simulink model "dcdc_zvs_full_bridge"  (R2026b)
settings: Solver=ode23tb  StopTime=simlength  FixedStep=tc  MaxStep=tc
values from neighbouring files (symbols this model uses):
  Idc_FS = max(Idab1_dc_nom,Idab2_dc_nom) * margin_factor    [init_model.m]
  L_core_length = 95    [magnetics_design_transformer.m]
  number_of_cells_2_sim = floor((Uout_nom-delta_load)/u_cell)    [init_model.m]    (also in run_sim_output_current_ctrl.m = floor((Uout_max-delta_load)/u_cell))
  Pnom = 175e3    (= 175000)    [init_model.m]
  tc = ts_dab/400    (= 5e-07)    [init_model.m]
  u_cell = 3.6    [init_model.m]
  Vdab2_dc_nom = ubattery2    (= 540)    [init_model.m]
  Vdc_FS = max(Vdab1_dc_nom,Vdab2_dc_nom) * margin_factor    [init_model.m]
libraries: fl_lib x32, nesl_utility x22, discrete_time_low_pass_filter x7, lithium_ion_battery x2, pi_ctrl x2, full_bridge_diode_rectifier x2, full_bridge_zvs_pwm_modulator x1, full_bridge_ideal_switch x1, full_bridge_igbt_based_with_thermal_model x1, full_bridge_mosfet_based_with_thermal_model_zvs x1, three_windings_transformer x1
(part 1 of 2)
settings Model: SimulationMode=accelerator  Creator=LTNBDA  LastModifiedBy=d.bagnara
settings SolverCC: AutoInsertRateTranBlk=on  SolverResetMethod=Robust  ZeroCrossAlgorithm=Adaptive  ZeroCrossControl=EnableAll
settings DataIOCC: DSMLogging=off  LimitDataPoints=on  MaxDataPoints=1  ReturnWorkspaceOutputs=off  SaveFormat=Array  SaveOutput=off  SaveTime=off  SignalLogging=off  SignalLoggingSaveFormat=ModelDataLogs
settings OptimizationCC: EfficientMapNaN2IntZero=off  LifeSpan=inf  MemsetInitFltsAndDblsToZero=off
settings DebuggingCC: ArithmeticOperatorsInVariantConditions=warning  FcnCallInpInsideContextMsg=warning  MergeDetectMultiDrivingBlocksExec=none  MultiTaskCondExecSysMsg=none  MultiTaskDSMMsg=warning  MultiTaskRateTransMsg=warning  SFNoUnconditionalDefaultTransitionDiag=warning  SFUnexpectedBacktrackingDiag=warning  SaveWithParameterizedLinksMsg=none  SignalResolutionControl=TryResolveAllWithWarning  SolverPrmCheckMsg=warning  StateNameClashWarn=warning  UnderspecifiedInitializationDetection=Classic
settings HardwareCC: ProdEndianess=Unspecified  ProdEqTarget=off  ProdHWDeviceType=Generic->64-bit Embedded Processor (LP64)  ProdIntDivRoundTo=Undefined  ProdLargestAtomicFloat=None  TargetEndianess=LittleEndian  TargetHWDeviceType=MATLAB Host  TargetIntDivRoundTo=Zero  TargetLongLongMode=on
settings ModelReferenceCC: PropagateSignalLabelsOutOfModel=off
settings SFSimCC: CustomCodeUndefinedFunction=UseInterfaceOnly  SimUseLocalCustomCode=off
settings RTWCC: RTWUseLocalCustomCode=off
settings CodeAppCC: StateflowObjectComments=on
settings GRTTargetCC: CombineOutputUpdateFcns=off  GRTInterface=on  TargetLangStandard=C89/C90 (ANSI)
settings ConfigComp: CovExternalEMLEnable=off  CovSaveCumulativeToWorkspaceVar=on  CovSaveSingleToWorkspaceVar=on
settings SimscapeCC: SimscapeNormalizeSystem=off  SimscapeUseEnergyAccounting=off

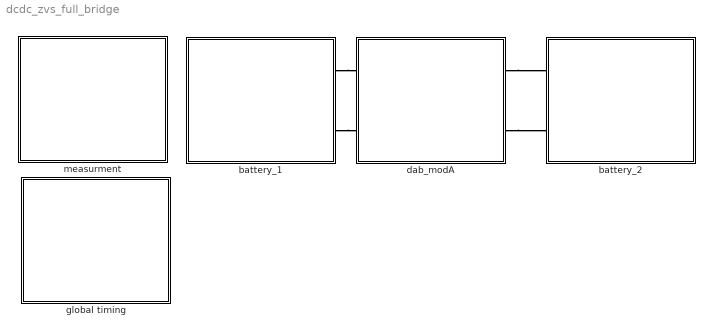
== system dcdc_zvs_full_bridge ==
  battery_1 : Subsystem
  battery_2 : Subsystem
  dab_modA : Subsystem
  global timing : Subsystem
  measurment : Subsystem
  connections:
  dab_modA/RConn2 -- battery_2/RConn2
  dab_modA/RConn1 -- battery_2/RConn1
  battery_1/RConn1 -- dab_modA/LConn1
  battery_1/RConn2 -- dab_modA/LConn2

== system dcdc_zvs_full_bridge/battery_1 ==
  Electrical Reference1 : fl_lib/Electrical/Electrical Elements/Electrical Reference
  Solver Configuration : nesl_utility/Solver Configuration  PhysicalDomain=network_engine_domain  SubClassName=solver  LeftPortType=input  RightPortType=generic  Tones=[]  Harmonics=[]  SimulateNoise=off  Profile=off  UseLocalSampling=off  EnableSwitchedLinearOptims=on  FrequencyDomain=off  UseCCode=off  RelTol=0.001  AbsTol=0.001  MinStep=1e-09  ToWorkspace=off  RevertToSquareIcSolve=off  NumHomotopyIterations=100  PhasorMode=off  PhasorModeNumHarmonics=1  ConsistencySolver=NEWTON_FTOL  CanonicalOrdering=UNORDERED  OptimizeIntermediates=UNOPTIMIZED  MulticoreSolverChoice=BACKWARD_EULER  IndexReductionMethod=DerivativeReplacement  DoDC=off  ResidualTolerance=1e-09  ConsistencyTolSource=GLOBAL  ConsistencyAbsTol=0.001  ConsistencyRelTol=0.001  ConsistencyTolFactor=0.001  UseLocalSolver=on  LocalSolverChoice=NE_BACKWARD_EULER_ADVANCER  ResolveIndetEquations=on  FunctionEvalNumThread=1  LocalSolverSampleTime=tc  DoFixedCost=on  MaxNonlinIter=5  MaxModeIter=2  ComputeImpulses=off  ImpulseIterations=2  LinearAlgebra=auto  LinearAlgebraNumThread=0  EquationFormulation=NE_TIME_EF  DelaysMemoryBudget=1024  AutomaticFiltering=on  FilteringTimeConstant=0.001  PartitionStorageMethod=AS_NEEDED  PartitionMemoryBudget=1024  PartitionMethod=BALANCED  MultibodyUseLocalSolver=off  MultibodyLocalSolverChoice=ODE1  MultibodyLocalSolverSampleTime=0.001
  litium ion battery 1 : Scope
      settings: ActiveDisplayYMinimum=741.26003825137309  ActiveDisplayYMaximum=832.30459900669575  DataLoggingVariableName=ScopeData3
  litium_ion_battery_1 : lithium_ion_battery/lithium_ion_battery  Q=Q  number_of_cells=number_of_cells_1_sim  E_1=E_1  E0=E0  E1=E1  E2=E2  E3=E3  Elog=Elog  R0=R0  R1=R1  C1=C1  M=M  alpha=alpha  soc_init=soc_init  ts_battery=ts_battery  q1Kalman=q1Kalman  q2Kalman=q2Kalman  q3Kalman=q3Kalman  rKalman=rKalman  tc=tc  enable_white_noise_m=0  battery_voltage_init_m=750
  single_phase_ui_measure : Subsystem
  dc+ : PMIOPort  Side=Right
  dc- : PMIOPort  Port=2  Side=Right
  wires:
  litium_ion_battery_1/1 -> litium ion battery 1/1
  connections:
  litium_ion_battery_1/RConn2 -- single_phase_ui_measure/LConn2 -- Electrical Reference1/LConn1 -- Solver Configuration/RConn1
  single_phase_ui_measure/RConn1 -- dc+/RConn1
  single_phase_ui_measure/LConn1 -- litium_ion_battery_1/RConn1
  dc-/RConn1 -- single_phase_ui_measure/RConn2

== system dcdc_zvs_full_bridge/battery_2 ==
  Electrical Reference1 : fl_lib/Electrical/Electrical Elements/Electrical Reference
  Resistor : fl_lib/Electrical/Electrical Elements/Resistor  Commented=on  R=(number_of_cells_2_sim*u_cell)^2/Pnom Ohm  i_specify=off  i_priority=None  i=0 A  i_nominal_specify=off  i_nominal_value=1  i_nominal_unit=A  v_specify=off  v_priority=None  v=0 V  v_nominal_specify=off  v_nominal_value=1  v_nominal_unit=V
  lithium_ion_battery_2 : lithium_ion_battery/lithium_ion_battery  Q=Q  number_of_cells=number_of_cells_2_sim  E_1=E_1  E0=E0  E1=E1  E2=E2  E3=E3  Elog=Elog  R0=R0  R1=R1  C1=C1  M=M  alpha=alpha  soc_init=soc_init  ts_battery=ts_battery  q1Kalman=q1Kalman  q2Kalman=q2Kalman  q3Kalman=q3Kalman  rKalman=rKalman  tc=tc  enable_white_noise_m=0  battery_voltage_init_m=750
  litium ion battery 2 : Scope
      settings: ActiveDisplayYMinimum=-504.55573672544915  ActiveDisplayYMaximum=-53.228038634989844  DataLoggingVariableName=ScopeData3
  single_phase_ui_measure : Subsystem
  dc+ : PMIOPort  Side=Right
  dc- : PMIOPort  Port=2  Side=Right
  wires:
  lithium_ion_battery_2/1 -> litium ion battery 2/1
  connections:
  dc-/RConn1 -- single_phase_ui_measure/RConn2
  lithium_ion_battery_2/RConn1 -- single_phase_ui_measure/LConn1 -- Resistor/LConn1
  single_phase_ui_measure/RConn1 -- dc+/RConn1
  Electrical Reference1/LConn1 -- single_phase_ui_measure/LConn2 -- Resistor/RConn1 -- lithium_ion_battery_2/RConn2

== system dcdc_zvs_full_bridge/dab_modA ==
  dab_ctrl : Subsystem
  dcdc_with_galvanic_isolation : Subsystem
  udc(+) : PMIOPort  Side=Right
  udc(-) : PMIOPort  Port=2  Side=Right
  dc+ : PMIOPort  Port=3  Side=Left
  dc- : PMIOPort  Port=4  Side=Left
  wires:
  dab_ctrl/1(gate_commands) -> dcdc_with_galvanic_isolation/1(gate_commands)
  connections:
  udc(+)/RConn1 -- dcdc_with_galvanic_isolation/RConn1
  udc(-)/RConn1 -- dcdc_with_galvanic_isolation/RConn2
  dc-/RConn1 -- dcdc_with_galvanic_isolation/LConn2
  dc+/RConn1 -- dcdc_with_galvanic_isolation/LConn1

== system dcdc_zvs_full_bridge/global timing ==
  Unit Delay : UnitDelay  SampleTime=tc
  time_afe1 : Subsystem  mask{k=1}
      mask prompts: k "Time Gain"
      mask Display:
      | disp('time-gen');
      | port_label('input', 1, 'crt');
      | port_label('output', 1, 'tout');
  time_afe3 : Subsystem  mask{k=1}
      mask prompts: k "Time Gain"
      mask Display:
      | disp('time-gen');
      | port_label('output', 1, 'tout');
  tag scope: time_dab_module_1=global, time_master=global
  wires:
  time_afe1/1(Out1) -> [time_dab_module_1]
  time_afe3/1(Out1) -> [time_master]
  [local_time_corr_dcdc1] -> Unit Delay/1
  Unit Delay/1 -> time_afe1/1(correction_time)

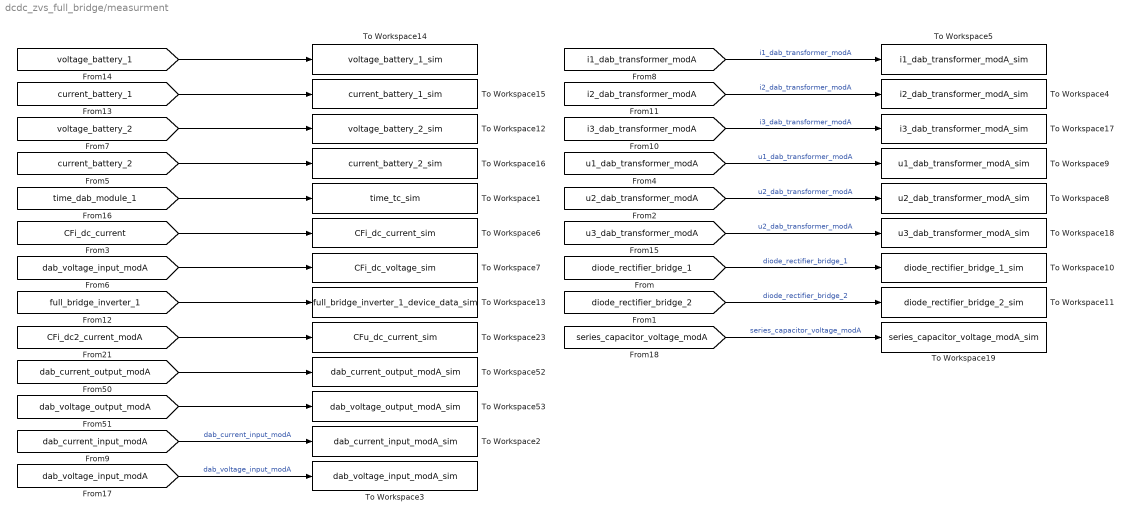
== system dcdc_zvs_full_bridge/measurment ==
  To Workspace1 : ToWorkspace  VariableName=time_tc_sim  SampleTime=tc
      settings: MaxDataPoints=Nc
  To Workspace10 : ToWorkspace  VariableName=diode_rectifier_bridge_1_sim  SampleTime=tc
      settings: MaxDataPoints=Nc
  To Workspace11 : ToWorkspace  VariableName=diode_rectifier_bridge_2_sim  SampleTime=tc
      settings: MaxDataPoints=Nc
  To Workspace12 : ToWorkspace  VariableName=voltage_battery_2_sim  SampleTime=tc
      settings: MaxDataPoints=Nc
  To Workspace13 : ToWorkspace  VariableName=full_bridge_inverter_1_device_data_sim  SampleTime=tc
      settings: MaxDataPoints=Nc
  To Workspace14 : ToWorkspace  VariableName=voltage_battery_1_sim  SampleTime=tc
      settings: MaxDataPoints=Nc
  To Workspace15 : ToWorkspace  VariableName=current_battery_1_sim  SampleTime=tc
      settings: MaxDataPoints=Nc
  To Workspace16 : ToWorkspace  VariableName=current_battery_2_sim  SampleTime=tc
      settings: MaxDataPoints=Nc
  To Workspace17 : ToWorkspace  VariableName=i3_dab_transformer_modA_sim  SampleTime=tc
      settings: MaxDataPoints=Nc
  To Workspace18 : ToWorkspace  VariableName=u3_dab_transformer_modA_sim  SampleTime=tc
      settings: MaxDataPoints=Nc
  To Workspace19 : ToWorkspace  VariableName=series_capacitor_voltage_modA_sim  SampleTime=tc
      settings: MaxDataPoints=Nc
  To Workspace2 : ToWorkspace  VariableName=dab_current_input_modA_sim  SampleTime=tc
      settings: MaxDataPoints=Nc
  To Workspace23 : ToWorkspace  VariableName=CFu_dc_current_sim  SampleTime=tc
      settings: MaxDataPoints=Nc
  To Workspace3 : ToWorkspace  VariableName=dab_voltage_input_modA_sim  SampleTime=tc
      settings: MaxDataPoints=Nc
  To Workspace4 : ToWorkspace  VariableName=i2_dab_transformer_modA_sim  SampleTime=tc
      settings: MaxDataPoints=Nc
  To Workspace5 : ToWorkspace  VariableName=i1_dab_transformer_modA_sim  SampleTime=tc
      settings: MaxDataPoints=Nc
  To Workspace52 : ToWorkspace  VariableName=dab_current_output_modA_sim  SampleTime=tc
      settings: MaxDataPoints=Nc
  To Workspace53 : ToWorkspace  VariableName=dab_voltage_output_modA_sim  SampleTime=tc
      settings: MaxDataPoints=Nc
  To Workspace6 : ToWorkspace  VariableName=CFi_dc_current_sim  SampleTime=tc
      settings: MaxDataPoints=Nc
  To Workspace7 : ToWorkspace  VariableName=CFi_dc_voltage_sim  SampleTime=tc
      settings: MaxDataPoints=Nc
  To Workspace8 : ToWorkspace  VariableName=u2_dab_transformer_modA_sim  SampleTime=tc
      settings: MaxDataPoints=Nc
  To Workspace9 : ToWorkspace  VariableName=u1_dab_transformer_modA_sim  SampleTime=tc
      settings: MaxDataPoints=Nc
  wires:
  [time_dab_module_1] -> To Workspace1/1
  [CFi_dc_current] -> To Workspace6/1
  [dab_voltage_input_modA] -> To Workspace7/1
  [voltage_battery_1] -> To Workspace14/1
  [current_battery_1] -> To Workspace15/1
  [CFi_dc2_current_modA] -> To Workspace23/1
  [dab_voltage_output_modA] -> To Workspace53/1
  [dab_current_output_modA] -> To Workspace52/1
  [full_bridge_inverter_1] -> To Workspace13/1
  [dab_current_input_modA] -> To Workspace2/1  "dab_current_input_modA"
  [dab_voltage_input_modA] -> To Workspace3/1  "dab_voltage_input_modA"
  [i2_dab_transformer_modA] -> To Workspace4/1  "i2_dab_transformer_modA"
  [i1_dab_transformer_modA] -> To Workspace5/1  "i1_dab_transformer_modA"
  [u2_dab_transformer_modA] -> To Workspace8/1  "u2_dab_transformer_modA"
  [u1_dab_transformer_modA] -> To Workspace9/1  "u1_dab_transformer_modA"
  [voltage_battery_2] -> To Workspace12/1
  [current_battery_2] -> To Workspace16/1
  [diode_rectifier_bridge_1] -> To Workspace10/1  "diode_rectifier_bridge_1"
  [diode_rectifier_bridge_2] -> To Workspace11/1  "diode_rectifier_bridge_2"
  [i3_dab_transformer_modA] -> To Workspace17/1  "i3_dab_transformer_modA"
  [u3_dab_transformer_modA] -> To Workspace18/1  "u2_dab_transformer_modA"
  [series_capacitor_voltage_modA] -> To Workspace19/1  "series_capacitor_voltage_modA"

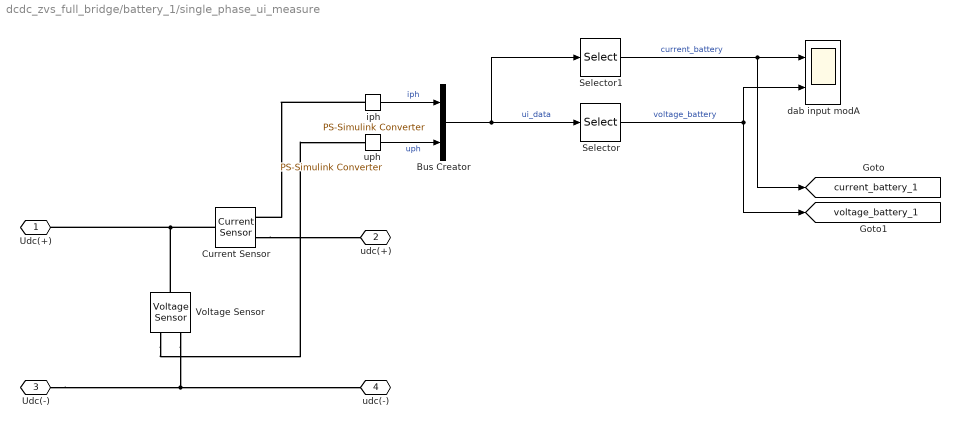
== system dcdc_zvs_full_bridge/battery_1/single_phase_ui_measure ==
  Bus Creator : BusCreator  Inputs=2
  Current Sensor : fl_lib/Electrical/Electrical Sensors/Current Sensor
  Selector : Selector  InputPortWidth=2  IndexOptions=Index vector (dialog)  Indices=2  OutputSizes=1  RuntimeRangeChecks=off
  Selector1 : Selector  InputPortWidth=2  IndexOptions=Index vector (dialog)  Indices=1  OutputSizes=1  RuntimeRangeChecks=off
  Voltage Sensor : fl_lib/Electrical/Electrical Sensors/Voltage Sensor
  dab input modA : Scope  NumInputPorts=2
      settings: SampleTime=tc  ActiveDisplayYMinimum=-4428.9106738971032  ActiveDisplayYMaximum=4853.7975894934307  DataLoggingVariableName=ScopeData2
  iph : nesl_utility/PS-Simulink Converter  PhysicalDomain=network_engine_domain  SubClassName=ps_output  LeftPortType=input  RightPortType=output  PseudoPeriodic=off  Frequencies=[]  VectorFormat=1-D array  Unit=A  AffineConversion=off
  uph : nesl_utility/PS-Simulink Converter  PhysicalDomain=network_engine_domain  SubClassName=ps_output  LeftPortType=input  RightPortType=output  PseudoPeriodic=off  Frequencies=[]  VectorFormat=1-D array  Unit=V  AffineConversion=off
  Udc(+) : PMIOPort  Side=Left
  udc(+) : PMIOPort  Port=2  Side=Right
  Udc(-) : PMIOPort  Port=3  Side=Left
  udc(-) : PMIOPort  Port=4  Side=Right
  tag scope: current_battery_1=global, voltage_battery_1=global
  wires:
  Bus Creator/1 -> Selector/1, Selector1/1  "ui_data"
  iph/1 -> Bus Creator/1  "iph"
  uph/1 -> Bus Creator/2  "uph"
  Selector1/1 -> [current_battery_1], dab input modA/1  "current_battery"
  Selector/1 -> dab input modA/2, [voltage_battery_1]  "voltage_battery"
  connections:
  iph/LConn1 -- Current Sensor/RConn1
  Voltage Sensor/LConn1 -- Current Sensor/LConn1 -- Udc(+)/RConn1
  Current Sensor/RConn2 -- udc(+)/RConn1
  Voltage Sensor/RConn1 -- uph/LConn1
  Voltage Sensor/RConn2 -- Udc(-)/RConn1 -- udc(-)/RConn1

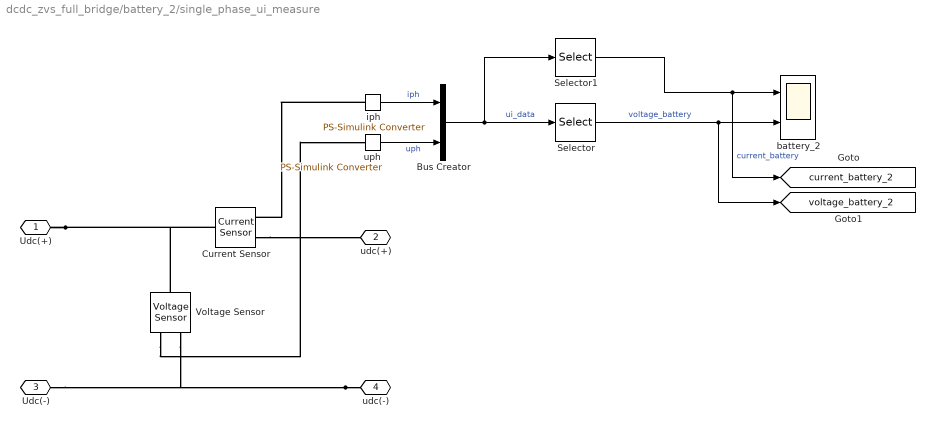
== system dcdc_zvs_full_bridge/battery_2/single_phase_ui_measure ==
  Bus Creator : BusCreator  Inputs=2
  Current Sensor : fl_lib/Electrical/Electrical Sensors/Current Sensor
  Selector : Selector  InputPortWidth=2  IndexOptions=Index vector (dialog)  Indices=2  OutputSizes=1  RuntimeRangeChecks=off
  Selector1 : Selector  InputPortWidth=2  IndexOptions=Index vector (dialog)  Indices=1  OutputSizes=1  RuntimeRangeChecks=off
  Voltage Sensor : fl_lib/Electrical/Electrical Sensors/Voltage Sensor
  battery_2 : Scope  NumInputPorts=2
      settings: SampleTime=tc  ActiveDisplayYMinimum=-384.09444656466405  ActiveDisplayYMaximum=-245.67258584008431  DataLoggingVariableName=ScopeData2
  iph : nesl_utility/PS-Simulink Converter  PhysicalDomain=network_engine_domain  SubClassName=ps_output  LeftPortType=input  RightPortType=output  PseudoPeriodic=off  Frequencies=[]  VectorFormat=1-D array  Unit=A  AffineConversion=off
  uph : nesl_utility/PS-Simulink Converter  PhysicalDomain=network_engine_domain  SubClassName=ps_output  LeftPortType=input  RightPortType=output  PseudoPeriodic=off  Frequencies=[]  VectorFormat=1-D array  Unit=V  AffineConversion=off
  Udc(+) : PMIOPort  Side=Left
  udc(+) : PMIOPort  Port=2  Side=Right
  Udc(-) : PMIOPort  Port=3  Side=Left
  udc(-) : PMIOPort  Port=4  Side=Right
  tag scope: current_battery_2=global, voltage_battery_2=global
  wires:
  Selector/1 -> [voltage_battery_2], battery_2/2  "voltage_battery"
  Selector1/1 -> battery_2/1, [current_battery_2]  "current_battery"
  uph/1 -> Bus Creator/2  "uph"
  iph/1 -> Bus Creator/1  "iph"
  Bus Creator/1 -> Selector1/1, Selector/1  "ui_data"
  connections:
  udc(-)/RConn1 -- Udc(-)/RConn1 -- Voltage Sensor/RConn2
  Voltage Sensor/RConn1 -- uph/LConn1
  Current Sensor/RConn2 -- udc(+)/RConn1
  Udc(+)/RConn1 -- Current Sensor/LConn1 -- Voltage Sensor/LConn1
  iph/LConn1 -- Current Sensor/RConn1

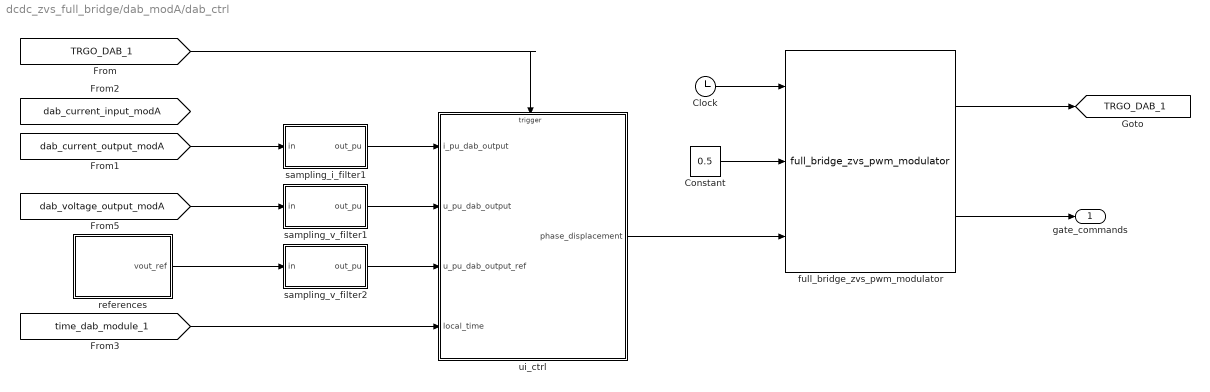
== system dcdc_zvs_full_bridge/dab_modA/dab_ctrl ==
  Clock : Clock
  Constant : Constant  Value=0.5
  full_bridge_zvs_pwm_modulator : full_bridge_zvs_pwm_modulator/full_bridge_zvs_pwm_modulator  fPWM_m=fPWM_DAB  m_up_m=1  m_low_m=0  dead_time_DAB_m=dead_time_DAB  pos_cmd_gate_m=15  neg_cmd_gate_m=-10  polarity_m=1  tc_m=tc  max_phase_displacement_m=pi  trgo_double_update_m=TRGO_double_update
  references : Subsystem
  sampling_i_filter1 : Subsystem
  sampling_v_filter1 : Subsystem
  sampling_v_filter2 : Subsystem
  ui_ctrl : Subsystem
  gate_commands : Outport
  tag scope: TRGO_DAB_1=global
  wires:
  [dab_voltage_output_modA] -> sampling_v_filter1/1(in)
  sampling_i_filter1/1(out_pu) -> ui_ctrl/1(i_pu_dab_output)
  sampling_v_filter1/1(out_pu) -> ui_ctrl/2(u_pu_dab_output)
  sampling_v_filter2/1(out_pu) -> ui_ctrl/3(u_pu_dab_output_ref)
  references/1(vout_ref) -> sampling_v_filter2/1(in)
  full_bridge_zvs_pwm_modulator/2 -> gate_commands/1
  Clock/1 -> full_bridge_zvs_pwm_modulator/1
  full_bridge_zvs_pwm_modulator/1 -> [TRGO_DAB_1]
  [TRGO_DAB_1] -> ui_ctrl/Trigger
  Constant/1 -> full_bridge_zvs_pwm_modulator/2
  ui_ctrl/1(phase_displacement) -> full_bridge_zvs_pwm_modulator/3
  [dab_current_output_modA] -> sampling_i_filter1/1(in)
  [time_dab_module_1] -> ui_ctrl/4(local_time)

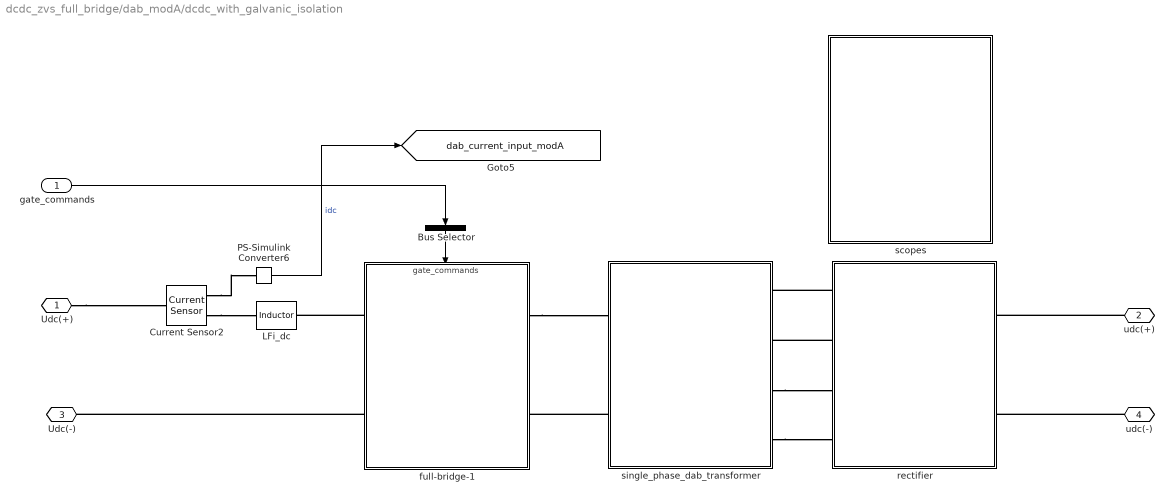
== system dcdc_zvs_full_bridge/dab_modA/dcdc_with_galvanic_isolation ==
  gate_commands : Inport
  Bus Selector : BusSelector  OutputSignals=gate_cmd_Q1,gate_cmd_Q2,gate_cmd_Q3,gate_cmd_Q4  OutputAsBus=on
  Current Sensor2 : fl_lib/Electrical/Electrical Sensors/Current Sensor
  LFi_dc : fl_lib/Electrical/Electrical Elements/Inductor  l=LFi_dc H  r=RLFi_dc Ohm  g=1e-9 1/Ohm  i_specify=off  i_priority=None  i=0 A  i_nominal_specify=off  i_nominal_value=1  i_nominal_unit=A  v_specify=off  v_priority=None  v=0 V  v_nominal_specify=off  v_nominal_value=1  v_nominal_unit=V  i_L_specify=off  i_L_priority=High  i_L=0 A  i_L_nominal_specify=off  i_L_nominal_value=1  i_L_nominal_unit=A
  PS-Simulink Converter6 : nesl_utility/PS-Simulink Converter  PhysicalDomain=network_engine_domain  SubClassName=ps_output  LeftPortType=input  RightPortType=output  PseudoPeriodic=off  Frequencies=[]  VectorFormat=1-D array  Unit=A  AffineConversion=on
  full-bridge-1 : Subsystem
      settings: PortSchema="{\"entries\":[{\"content\":{\"sides\":[{\"content\":{\"connectorIds\":[\"LConn1\",\"LConn2\"]},\"type\":\"ConnectorPlacement.EquallySpacedRectSide\",\"uuid\":\"c872503a-61af-4937-bdf2-4de4f8645573\"},{\"content\":{\"connectorIds\":[\"RConn1\",\"RConn2\"],\"side\":\"RIGHT\"},\"type\":\"ConnectorPlacement.EquallySpacedRectSide\",\"uuid\":\"3b83f060-86a2-4569-84b5-d9f7c0485347\"},{\"content\":{\"connectorIds\":[\"In1\"],\"side\":\"TOP\"},\"type\":\"ConnectorPlacement.EquallySpacedRectSide\",\"uuid\":\"bf191d46-ce71-4d15-9dd0-24cc57253577\"}]},\"type\":\"ConnectorPlacement.EquallySpacedConnector\",\"uuid\":\"1b28ceee-25d0-45ae-a3c4-c2563f0d63ba\"}],\"packageUris\":[\"http://schema.mathworks.com/mf0/Connector/R2020b\"],\"version\":\"1.0\"}"
  rectifier : Subsystem
  scopes : Subsystem
  single_phase_dab_transformer : Subsystem
  Udc(+) : PMIOPort  Side=Left
  udc(+) : PMIOPort  Port=2  Side=Right
  Udc(-) : PMIOPort  Port=3  Side=Left
  udc(-) : PMIOPort  Port=4  Side=Right
  tag scope: dab_current_input_modA=global
  wires:
  gate_commands/1 -> Bus Selector/1
  PS-Simulink Converter6/1 -> [dab_current_input_modA]  "idc"
  Bus Selector/1 -> full-bridge-1/1(gate_commands)
  connections:
  single_phase_dab_transformer/LConn2 -- full-bridge-1/LConn2
  full-bridge-1/RConn1 -- LFi_dc/RConn1
  full-bridge-1/RConn2 -- Udc(-)/RConn1
  full-bridge-1/LConn1 -- single_phase_dab_transformer/LConn1
  udc(-)/RConn1 -- rectifier/RConn2
  Current Sensor2/RConn2 -- LFi_dc/LConn1
  Udc(+)/RConn1 -- Current Sensor2/LConn1
  Current Sensor2/RConn1 -- PS-Simulink Converter6/LConn1
  rectifier/LConn1 -- single_phase_dab_transformer/RConn1
  rectifier/LConn2 -- single_phase_dab_transformer/RConn2
  udc(+)/RConn1 -- rectifier/RConn1
  single_phase_dab_transformer/RConn3 -- rectifier/LConn3
  single_phase_dab_transformer/RConn4 -- rectifier/LConn4

== system dcdc_zvs_full_bridge/global timing/time_afe1 ==
  correction_time : Inport
  Constant : Constant
  Gain : Gain  Gain=k
  Product : Product
  Sum : Sum  Inputs=|++
  time_1 : Clock
  Out1 : Outport
  wires:
  time_1/1 -> Gain/1
  Gain/1 -> Product/1
  Product/1 -> Out1/1
  correction_time/1 -> Sum/1
  Sum/1 -> Product/2
  Constant/1 -> Sum/2

== system dcdc_zvs_full_bridge/global timing/time_afe3 ==
  Gain : Gain  Gain=k
  time_1 : Clock
  Out1 : Outport
  wires:
  Gain/1 -> Out1/1
  time_1/1 -> Gain/1

== system dcdc_zvs_full_bridge/dab_modA/dab_ctrl/references ==
  Rate Limiter : RateLimiter  RisingSlewLimit=Vdab2_dc_nom*10  FallingSlewLimit=-Vdab2_dc_nom*10  SampleTimeMode=inherited
  Vout_dc_nom : Step  Time=1e-3  FinalValue=Vdab2_dc_nom  SampleTime=0
  vout_ref : Outport
  wires:
  Rate Limiter/1 -> vout_ref/1
  Vout_dc_nom/1 -> Rate Limiter/1

== system dcdc_zvs_full_bridge/dab_modA/dab_ctrl/sampling_i_filter1 ==
  in : Inport
  1/Ti3 : Gain  Gain=1/Idc_FS  OutDataTypeStr=double  SaturateOnIntegerOverflow=on  ParamDataTypeStr=Inherit: Same as input
  out_pu : Outport
  wires:
  in/1 -> 1/Ti3/1
  1/Ti3/1 -> out_pu/1

== system dcdc_zvs_full_bridge/dab_modA/dab_ctrl/sampling_v_filter1 ==
  in : Inport
  1/Ti3 : Gain  Gain=1/Vdc_FS  OutDataTypeStr=double  SaturateOnIntegerOverflow=on  ParamDataTypeStr=Inherit: Same as input
  out_pu : Outport
  wires:
  in/1 -> 1/Ti3/1
  1/Ti3/1 -> out_pu/1

== system dcdc_zvs_full_bridge/dab_modA/dab_ctrl/sampling_v_filter2 ==
  in : Inport
  1/Ti3 : Gain  Gain=1/Vdc_FS  OutDataTypeStr=double  SaturateOnIntegerOverflow=on  ParamDataTypeStr=Inherit: Same as input
  Saturation : Saturate  UpperLimit=1  LowerLimit=0  OutDataTypeStr=double
  out_pu : Outport
  wires:
  in/1 -> 1/Ti3/1
  1/Ti3/1 -> Saturation/1
  Saturation/1 -> out_pu/1

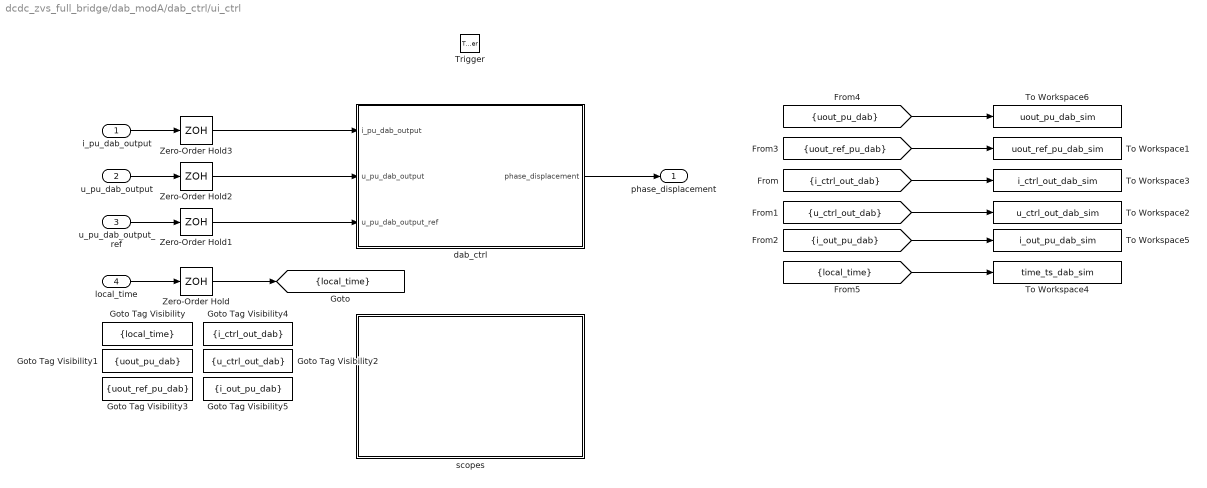
== system dcdc_zvs_full_bridge/dab_modA/dab_ctrl/ui_ctrl ==
  i_pu_dab_output : Inport
  u_pu_dab_output : Inport  Port=2
  u_pu_dab_output_ref : Inport  Port=3
  local_time : Inport  Port=4
  Trigger : TriggerPort  VariantControl=(inherit)  PortDimensions=1
  Goto Tag Visibility : GotoTagVisibility  GotoTag=local_time
  Goto Tag Visibility1 : GotoTagVisibility  GotoTag=uout_pu_dab
  Goto Tag Visibility2 : GotoTagVisibility  GotoTag=u_ctrl_out_dab
  Goto Tag Visibility3 : GotoTagVisibility  GotoTag=uout_ref_pu_dab
  Goto Tag Visibility4 : GotoTagVisibility  GotoTag=i_ctrl_out_dab
  Goto Tag Visibility5 : GotoTagVisibility  GotoTag=i_out_pu_dab
  To Workspace1 : ToWorkspace  VariableName=uout_ref_pu_dab_sim  SampleTime=-1
      settings: MaxDataPoints=Ns_dab
  To Workspace2 : ToWorkspace  VariableName=u_ctrl_out_dab_sim  SampleTime=-1
      settings: MaxDataPoints=Ns_dab
  To Workspace3 : ToWorkspace  VariableName=i_ctrl_out_dab_sim  SampleTime=-1
      settings: MaxDataPoints=Ns_dab
  To Workspace4 : ToWorkspace  VariableName=time_ts_dab_sim  SampleTime=-1
      settings: MaxDataPoints=Ns_dab
  To Workspace5 : ToWorkspace  VariableName=i_out_pu_dab_sim  SampleTime=-1
      settings: MaxDataPoints=Ns_dab
  To Workspace6 : ToWorkspace  VariableName=uout_pu_dab_sim  SampleTime=-1
      settings: MaxDataPoints=Ns_dab
  Zero-Order Hold{,1..3} (4 alike) : ZeroOrderHold  SampleTime=-1
  dab_ctrl : Subsystem
  scopes : Subsystem
  phase_displacement : Outport
  tag scope: local_time=scoped
  wires:
  i_pu_dab_output/1 -> Zero-Order Hold3/1
  u_pu_dab_output/1 -> Zero-Order Hold2/1
  u_pu_dab_output_ref/1 -> Zero-Order Hold1/1
  dab_ctrl/1(phase_displacement) -> phase_displacement/1
  local_time/1 -> Zero-Order Hold/1
  Zero-Order Hold1/1 -> dab_ctrl/3(u_pu_dab_output_ref)
  Zero-Order Hold2/1 -> dab_ctrl/2(u_pu_dab_output)
  Zero-Order Hold3/1 -> dab_ctrl/1(i_pu_dab_output)
  Zero-Order Hold/1 -> [local_time]
  [uout_ref_pu_dab] -> To Workspace1/1
  [uout_pu_dab] -> To Workspace6/1
  [u_ctrl_out_dab] -> To Workspace2/1
  [i_ctrl_out_dab] -> To Workspace3/1
  [local_time] -> To Workspace4/1
  [i_out_pu_dab] -> To Workspace5/1

== system dcdc_zvs_full_bridge/dab_modA/dcdc_with_galvanic_isolation/full-bridge-1 ==
  gate_commands : Inport
  dclink : Subsystem
  full-bridge ideal switch based : full_bridge_ideal_switch/full-bridge ideal switch based  Commented=on  Rds_on=Rds_on  Vdon_diode=Vdon_diode  Rdon_diode=Rdon_diode  Csnubber=Csnubber  Rsnubber=Rsnubber  Vth=Vth
  full-bridge-igbt-based-with-thermal-model : full_bridge_igbt_based_with_thermal_model/full-bridge-igbt-based-with-thermal-model  mass_heatsink_m=heatsink.no_weight  specific_heat_m=heatsink.cp  rth_mosfet_HA_m=heatsink.Rth_switch_HA  rth_mosfet_JH_m=dab.igbt.Rth_switch_JH  Rce_on_m=dab.igbt.Rce_on  Vce_sat_m=dab.igbt.Vce_sat  Vth_m=dab.igbt.Vth  Eon_m=dab.igbt.Eon  Eoff_m=dab.igbt.Eoff  Erec_m=dab.igbt.Erec  Voff_sw_loss_m=dab.igbt.Voff_sw_losses  Ion_sw_loss_m=dab.igbt.Ion_sw_losses  Vdon_diode_m=dab.igbt.Vdon_diode  Rdon_diode_m=dab.igbt.Rdon_diode  Csnubber_m=dab.igbt.Csnubber  Rsnubber_m=dab.igbt.Rsnubber  JunctionTermalMass_m=dab.igbt.JunctionTermalMass  Tambient_m=Tambient  DThs_init_m=DThs_init  filter_time_constant_m=dab.igbt.filter_time_constant  tc_m=tc
  full-bridge_mosfet_based_ with_thermal_model_zvs : full_bridge_mosfet_based_with_thermal_model_zvs/full-bridge_mosfet_based_ with_thermal_model_zvs  Commented=on  mass_heatsink_m=weigth  specific_heat_m=cp_al  rth_mosfet_HA_m=Rth_mosfet_HA  rth_mosfet_JH_m=dab_mosfet.Rth_mosfet_JH  Rds_on_m=dab_mosfet.Rds_on  Vth_m=dab_mosfet.Vth  Eon_m=dab_mosfet.Eon  Eoff_m=dab_mosfet.Eoff  Voff_sw_loss_m=dab_mosfet.Voff_sw_losses  Ion_sw_loss_m=dab_mosfet.Ion_sw_losses  Vdon_diode_m=dab_mosfet.Vdon_diode  Rdon_diode_m=dab_mosfet.Rdon_diode  JunctionTermalMass_m=dab_mosfet.JunctionTermalMass  Tambient_m=Tambient  DThs_init_m=DThs_init  Csnubber_m=dab_mosfet.Csnubber_zvs  Rsnubber_m=dab_mosfet.Rsnubber_zvs
  uac_1(+) : PMIOPort  Side=Left
  uac_1(-) : PMIOPort  Port=2  Side=Left
  Udc(+) : PMIOPort  Port=3  Side=Right
  Udc(-) : PMIOPort  Port=4  Side=Right
  tag scope: full_bridge_inverter_1=global
  wires:
  gate_commands/1 -> full-bridge ideal switch based/1, full-bridge-igbt-based-with-thermal-model/1, full-bridge_mosfet_based_ with_thermal_model_zvs/1
  full-bridge-igbt-based-with-thermal-model/1 -> [full_bridge_inverter_1]
  connections:
  uac_1(+)/RConn1 -- full-bridge_mosfet_based_ with_thermal_model_zvs/RConn1 -- full-bridge-igbt-based-with-thermal-model/RConn1 -- full-bridge ideal switch based/RConn1
  uac_1(-)/RConn1 -- full-bridge_mosfet_based_ with_thermal_model_zvs/RConn2 -- full-bridge-igbt-based-with-thermal-model/RConn2 -- full-bridge ideal switch based/RConn2
  dclink/LConn1 -- Udc(+)/RConn1
  dclink/RConn2 -- full-bridge ideal switch based/LConn2 -- full-bridge_mosfet_based_ with_thermal_model_zvs/LConn2 -- full-bridge-igbt-based-with-thermal-model/LConn2
  dclink/RConn1 -- full-bridge_mosfet_based_ with_thermal_model_zvs/LConn1 -- full-bridge-igbt-based-with-thermal-model/LConn1 -- full-bridge ideal switch based/LConn1
  dclink/LConn2 -- Udc(-)/RConn1

== system dcdc_zvs_full_bridge/dab_modA/dcdc_with_galvanic_isolation/rectifier ==
  dclink : Subsystem
  rectifier_1 : Subsystem
  rectifier_2 : Subsystem
  uac_2(+) : PMIOPort  Side=Left
  uac_2(-) : PMIOPort  Port=2  Side=Left
  udc(+) : PMIOPort  Port=3  Side=Right
  udc(-) : PMIOPort  Port=4  Side=Right
  uac_3(+) : PMIOPort  Port=5  Side=Left
  uac_3(-) : PMIOPort  Port=6  Side=Left
  connections:
  udc(+)/RConn1 -- dclink/RConn1
  udc(-)/RConn1 -- dclink/RConn2
  uac_2(+)/RConn1 -- rectifier_1/LConn1
  dclink/LConn1 -- rectifier_1/RConn1
  uac_2(-)/RConn1 -- rectifier_1/LConn2
  rectifier_2/LConn2 -- uac_3(-)/RConn1
  rectifier_2/LConn1 -- uac_3(+)/RConn1
  rectifier_1/RConn2 -- rectifier_2/RConn1
  rectifier_2/RConn2 -- dclink/LConn2

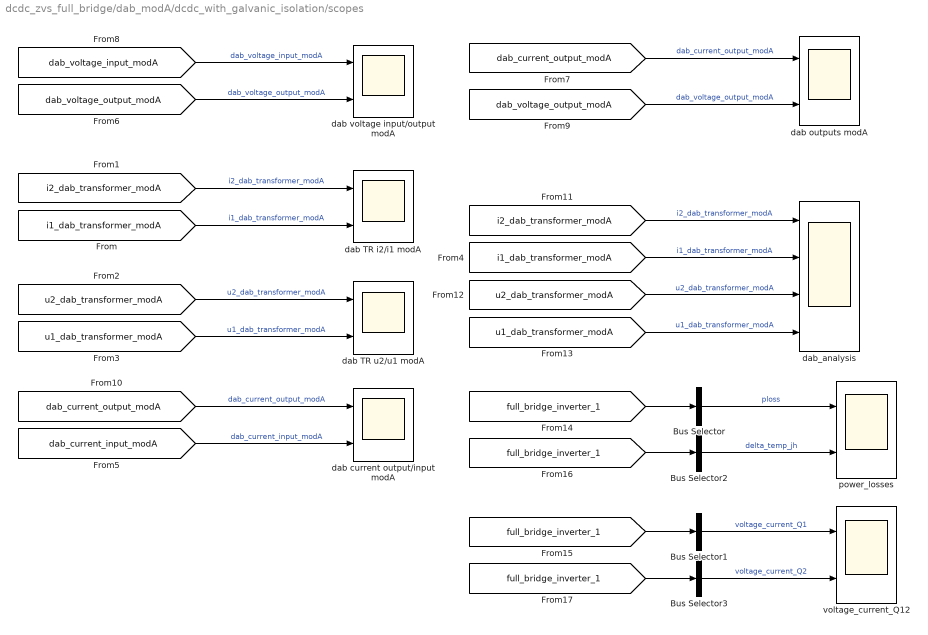
== system dcdc_zvs_full_bridge/dab_modA/dcdc_with_galvanic_isolation/scopes ==
  Bus Selector : BusSelector  OutputSignals=igbt_ploss_Q1,igbt_ploss_Q2,igbt_ploss_Q3,igbt_ploss_Q4  OutputAsBus=on
  Bus Selector1 : BusSelector  OutputSignals=igbt_voltage_Q1,igbt_current_Q1  OutputAsBus=on
  Bus Selector2 : BusSelector  OutputSignals=igbt_JH_temp_Q1,igbt_JH_temp_Q4,igbt_JH_temp_Q3,igbt_JH_temp_Q2  OutputAsBus=on
  Bus Selector3 : BusSelector  OutputSignals=igbt_voltage_Q2,igbt_current_Q2  OutputAsBus=on
  dab TR i2/i1 modA : Scope  NumInputPorts=2
      settings: SampleTime=tc  ActiveDisplayYMinimum=-1133.8385972087863  ActiveDisplayYMaximum=1130.02633442417  DataLoggingVariableName=ScopeData13
  dab TR u2/u1 modA : Scope  NumInputPorts=2
      settings: SampleTime=tc  ActiveDisplayYMinimum=-1550.0820677220172  ActiveDisplayYMaximum=1550.0802549877285  DataLoggingVariableName=ScopeData4
  dab current output/input modA : Scope  NumInputPorts=2
      settings: SampleTime=tc  ActiveDisplayYMinimum=-135.33312051034864  ActiveDisplayYMaximum=747.30464050791215  DataLoggingVariableName=ScopeData8
  dab outputs modA : Scope  NumInputPorts=2
      settings: SampleTime=tc  ActiveDisplayYMinimum=-176.23009288903958  ActiveDisplayYMaximum=438.21126312258008  DataLoggingVariableName=ScopeData6
  dab voltage input/output modA : Scope  NumInputPorts=2
      settings: SampleTime=tc  ActiveDisplayYMinimum=-220.62176138017153  ActiveDisplayYMaximum=1985.59585243125  DataLoggingVariableName=ScopeData10
  dab_analysis : Scope  NumInputPorts=4
      settings: SampleTime=tc  ActiveDisplayYMinimum=-3557.7801563621397  ActiveDisplayYMaximum=1974.1341111521624  DataLoggingVariableName=ScopeData5
  power_losses : Scope  NumInputPorts=2
      settings: SampleTime=tc  ActiveDisplayYMinimum=-425.00761228440524  ActiveDisplayYMaximum=-42.577893314830831
  voltage_current_Q12 : Scope  NumInputPorts=2
      settings: SampleTime=tc  ActiveDisplayYMinimum=251.19059945367908  ActiveDisplayYMaximum=349.10358624180844  DataLoggingVariableName=ScopeData14
  wires:
  [dab_voltage_input_modA] -> dab voltage input/output modA/1  "dab_voltage_input_modA"
  [dab_current_output_modA] -> dab current output/input modA/1  "dab_current_output_modA"
  [dab_voltage_output_modA] -> dab voltage input/output modA/2  "dab_voltage_output_modA"
  [dab_current_input_modA] -> dab current output/input modA/2  "dab_current_input_modA"
  [i2_dab_transformer_modA] -> dab TR i2/i1 modA/1  "i2_dab_transformer_modA"
  [i1_dab_transformer_modA] -> dab TR i2/i1 modA/2  "i1_dab_transformer_modA"
  [u2_dab_transformer_modA] -> dab TR u2/u1 modA/1  "u2_dab_transformer_modA"
  [u1_dab_transformer_modA] -> dab TR u2/u1 modA/2  "u1_dab_transformer_modA"
  [dab_voltage_output_modA] -> dab outputs modA/2  "dab_voltage_output_modA"
  [dab_current_output_modA] -> dab outputs modA/1  "dab_current_output_modA"
  [full_bridge_inverter_1] -> Bus Selector/1
  Bus Selector/1 -> power_losses/1  "ploss"
  Bus Selector2/1 -> power_losses/2  "delta_temp_jh"
  [full_bridge_inverter_1] -> Bus Selector2/1
  [u1_dab_transformer_modA] -> dab_analysis/4  "u1_dab_transformer_modA"
  [u2_dab_transformer_modA] -> dab_analysis/3  "u2_dab_transformer_modA"
  [i1_dab_transformer_modA] -> dab_analysis/2  "i1_dab_transformer_modA"
  [i2_dab_transformer_modA] -> dab_analysis/1  "i2_dab_transformer_modA"
  [full_bridge_inverter_1] -> Bus Selector3/1
  Bus Selector3/1 -> voltage_current_Q12/2  "voltage_current_Q2"
  Bus Selector1/1 -> voltage_current_Q12/1  "voltage_current_Q1"
  [full_bridge_inverter_1] -> Bus Selector1/1

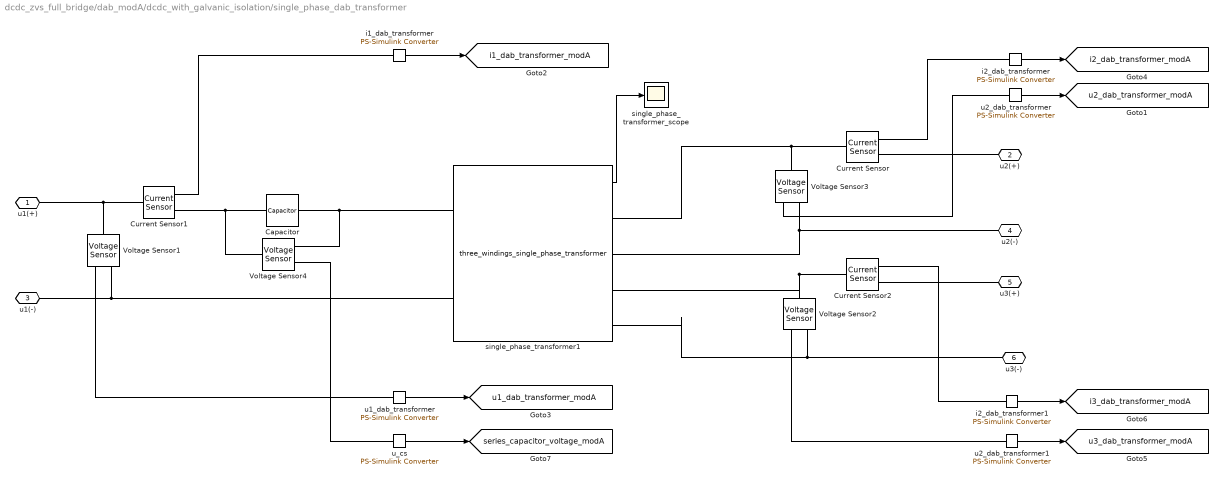
== system dcdc_zvs_full_bridge/dab_modA/dcdc_with_galvanic_isolation/single_phase_dab_transformer ==
  Capacitor : fl_lib/Electrical/Electrical Elements/Capacitor  c=Cs_dab F  r=1e-6 Ohm  g=0 1/Ohm  i_specify=off  i_priority=None  i=0 A  i_nominal_specify=off  i_nominal_value=1  i_nominal_unit=A  v_specify=off  v_priority=None  v=0 V  v_nominal_specify=off  v_nominal_value=1  v_nominal_unit=V  vc_specify=off  vc_priority=High  vc=0 V  vc_nominal_specify=off  vc_nominal_value=1  vc_nominal_unit=V
  Current Sensor : fl_lib/Electrical/Electrical Sensors/Current Sensor
  Current Sensor1 : fl_lib/Electrical/Electrical Sensors/Current Sensor
  Current Sensor2 : fl_lib/Electrical/Electrical Sensors/Current Sensor
  Voltage Sensor{1..4} (4 alike) : fl_lib/Electrical/Electrical Sensors/Voltage Sensor
  i1_dab_transformer : nesl_utility/PS-Simulink Converter  PhysicalDomain=network_engine_domain  SubClassName=ps_output  LeftPortType=input  RightPortType=output  PseudoPeriodic=off  Frequencies=[]  VectorFormat=1-D array  Unit=A  AffineConversion=off
  i2_dab_transformer : nesl_utility/PS-Simulink Converter  PhysicalDomain=network_engine_domain  SubClassName=ps_output  LeftPortType=input  RightPortType=output  PseudoPeriodic=off  Frequencies=[]  VectorFormat=1-D array  Unit=A  AffineConversion=off
  i2_dab_transformer1 : nesl_utility/PS-Simulink Converter  PhysicalDomain=network_engine_domain  SubClassName=ps_output  LeftPortType=input  RightPortType=output  PseudoPeriodic=off  Frequencies=[]  VectorFormat=1-D array  Unit=A  AffineConversion=off
  single_phase_transformer1 : three_windings_transformer/three_windings_single_phase_transformer  lm_trafo=lm_trafo  m1=m1  m2=m2  m3=m3  rd1_trafo=rd1_trafo  rd2_trafo=rd2_trafo  rd3_trafo=rd3_trafo  ld1_trafo=ld1_trafo  ld2_trafo=ld2_trafo  ld3_trafo=ld3_trafo  rfe_trafo=rfe_trafo  length_core=L_core_length/100  mu0=mu0  mur=mur
  single_phase_transformer_scope : Scope
      settings: DataLoggingVariableName=ScopeData9
  u1_dab_transformer : nesl_utility/PS-Simulink Converter  PhysicalDomain=network_engine_domain  SubClassName=ps_output  LeftPortType=input  RightPortType=output  PseudoPeriodic=off  Frequencies=[]  VectorFormat=1-D array  Unit=V  AffineConversion=on
  u2_dab_transformer : nesl_utility/PS-Simulink Converter  PhysicalDomain=network_engine_domain  SubClassName=ps_output  LeftPortType=input  RightPortType=output  PseudoPeriodic=off  Frequencies=[]  VectorFormat=1-D array  Unit=V  AffineConversion=on
  u2_dab_transformer1 : nesl_utility/PS-Simulink Converter  PhysicalDomain=network_engine_domain  SubClassName=ps_output  LeftPortType=input  RightPortType=output  PseudoPeriodic=off  Frequencies=[]  VectorFormat=1-D array  Unit=V  AffineConversion=on
  u_cs : nesl_utility/PS-Simulink Converter  PhysicalDomain=network_engine_domain  SubClassName=ps_output  LeftPortType=input  RightPortType=output  PseudoPeriodic=off  Frequencies=[]  VectorFormat=1-D array  Unit=V  AffineConversion=on
  u1(+) : PMIOPort  Side=Left
  u2(+) : PMIOPort  Port=2  Side=Right
  u1(-) : PMIOPort  Port=3  Side=Left
  u2(-) : PMIOPort  Port=4  Side=Right
  u3(+) : PMIOPort  Port=5  Side=Right
  u3(-) : PMIOPort  Port=6  Side=Right
  tag scope: i1_dab_transformer_modA=global, i2_dab_transformer_modA=global, i3_dab_transformer_modA=global, series_capacitor_voltage_modA=global, u1_dab_transformer_modA=global, u2_dab_transformer_modA=global, u3_dab_transformer_modA=global
  wires:
  i2_dab_transformer/1 -> [i2_dab_transformer_modA]
  u2_dab_transformer/1 -> [u2_dab_transformer_modA]
  u1_dab_transformer/1 -> [u1_dab_transformer_modA]
  i1_dab_transformer/1 -> [i1_dab_transformer_modA]
  single_phase_transformer1/1 -> single_phase_transformer_scope/1
  u2_dab_transformer1/1 -> [u3_dab_transformer_modA]
  i2_dab_transformer1/1 -> [i3_dab_transformer_modA]
  u_cs/1 -> [series_capacitor_voltage_modA]
  connections:
  Current Sensor/RConn2 -- u2(+)/RConn1
  Voltage Sensor3/RConn2 -- single_phase_transformer1/RConn2 -- u2(-)/RConn1
  Current Sensor/RConn1 -- i2_dab_transformer/LConn1
  u1(-)/RConn1 -- single_phase_transformer1/LConn2 -- Voltage Sensor1/RConn2
  Current Sensor1/LConn1 -- u1(+)/RConn1 -- Voltage Sensor1/LConn1
  Voltage Sensor1/RConn1 -- u1_dab_transformer/LConn1
  Current Sensor1/RConn1 -- i1_dab_transformer/LConn1
  Current Sensor/LConn1 -- single_phase_transformer1/RConn1 -- Voltage Sensor3/LConn1
  u2_dab_transformer/LConn1 -- Voltage Sensor3/RConn1
  single_phase_transformer1/LConn1 -- Voltage Sensor4/RConn2 -- Capacitor/RConn1
  Voltage Sensor2/RConn2 -- single_phase_transformer1/RConn4 -- u3(-)/RConn1
  Current Sensor2/LConn1 -- Voltage Sensor2/LConn1 -- single_phase_transformer1/RConn3
  u2_dab_transformer1/LConn1 -- Voltage Sensor2/RConn1
  Current Sensor2/RConn1 -- i2_dab_transformer1/LConn1
  Current Sensor2/RConn2 -- u3(+)/RConn1
  Capacitor/LConn1 -- Voltage Sensor4/LConn1 -- Current Sensor1/RConn2
  Voltage Sensor4/RConn1 -- u_cs/LConn1

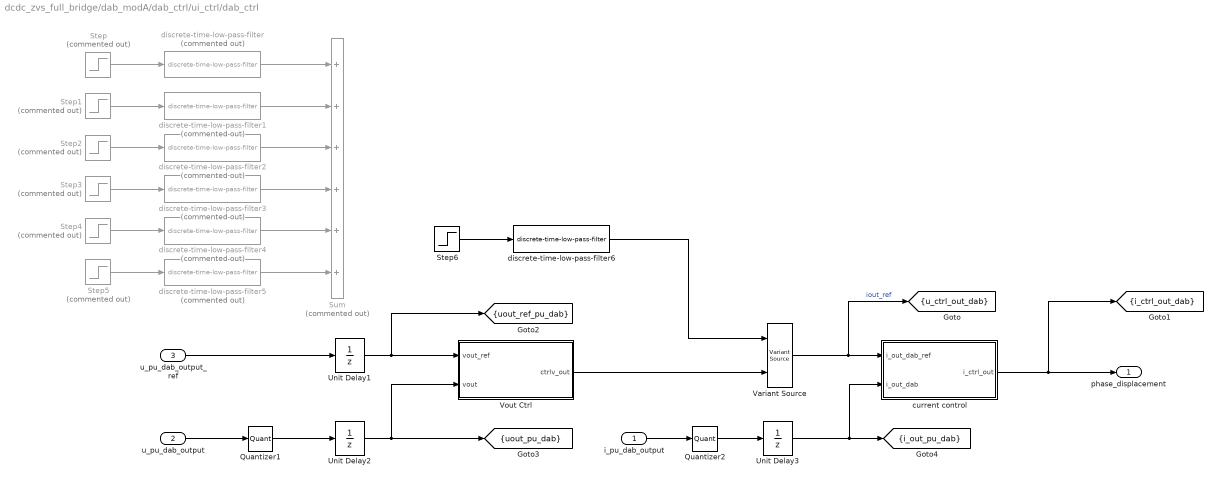
== system dcdc_zvs_full_bridge/dab_modA/dab_ctrl/ui_ctrl/dab_ctrl ==
  i_pu_dab_output : Inport
  u_pu_dab_output : Inport  Port=2
  u_pu_dab_output_ref : Inport  Port=3
  Quantizer1 : Quantizer  QuantizationInterval=adc12_quantization
  Quantizer2 : Quantizer  QuantizationInterval=adc12_quantization
  Step : Step  Commented=on  Time=0.05  FinalValue=0.25
  Step1 : Step  Commented=on  Time=0.4  FinalValue=0.75
  Step2 : Step  Commented=on  Time=0.6  FinalValue=0.25
  Step3 : Step  Commented=on  Time=0.8  FinalValue=-1
  Step4 : Step  Commented=on  FinalValue=-0.75
  Step5 : Step  Commented=on  Time=1.25  FinalValue=-0.5
  Step6 : Step  Time=0.25  InitialValue=0.25  FinalValue=i_out_dab_pu_ref_1
  Sum : Sum  Commented=on  Inputs=++++++
  Unit Delay1 : UnitDelay  SampleTime=-1
  Unit Delay2 : UnitDelay  SampleTime=-1
  Unit Delay3 : UnitDelay  SampleTime=-1
  Variant Source : VariantSource  VariantControls={true, false}
  Vout Ctrl : Subsystem
  current control : Subsystem
  discrete-time-low-pass-filter{,1..5} (6 alike) : discrete_time_low_pass_filter/discrete-time-low-pass-filter  Commented=on  tau=0.02  ts=ts_dab
  discrete-time-low-pass-filter6 : discrete_time_low_pass_filter/discrete-time-low-pass-filter  tau=0.02  ts=ts_dab
  phase_displacement : Outport
  tag scope: i_ctrl_out_dab=scoped, i_out_pu_dab=scoped, u_ctrl_out_dab=scoped, uout_pu_dab=scoped, uout_ref_pu_dab=scoped
  wires:
  Vout Ctrl/1(ctrlv_out) -> Variant Source/2
  Variant Source/1 -> [u_ctrl_out_dab], current control/1(i_out_dab_ref)  "iout_ref"
  i_pu_dab_output/1 -> Quantizer2/1
  current control/1(i_ctrl_out) -> phase_displacement/1, [i_ctrl_out_dab]
  Unit Delay3/1 -> current control/2(i_out_dab), [i_out_pu_dab]
  Unit Delay2/1 -> [uout_pu_dab], Vout Ctrl/2(vout)
  Unit Delay1/1 -> Vout Ctrl/1(vout_ref), [uout_ref_pu_dab]
  u_pu_dab_output/1 -> Quantizer1/1
  Step/1 -> discrete-time-low-pass-filter/1
  Step1/1 -> discrete-time-low-pass-filter1/1
  Step2/1 -> discrete-time-low-pass-filter2/1
  Step3/1 -> discrete-time-low-pass-filter3/1
  Step4/1 -> discrete-time-low-pass-filter4/1
  Step5/1 -> discrete-time-low-pass-filter5/1
  discrete-time-low-pass-filter/1 -> Sum/1
  discrete-time-low-pass-filter1/1 -> Sum/2
  discrete-time-low-pass-filter2/1 -> Sum/3
  discrete-time-low-pass-filter3/1 -> Sum/4
  discrete-time-low-pass-filter4/1 -> Sum/5
  discrete-time-low-pass-filter5/1 -> Sum/6
  u_pu_dab_output_ref/1 -> Unit Delay1/1
  Quantizer1/1 -> Unit Delay2/1
  Quantizer2/1 -> Unit Delay3/1
  Step6/1 -> discrete-time-low-pass-filter6/1
  discrete-time-low-pass-filter6/1 -> Variant Source/1

== system dcdc_zvs_full_bridge/dab_modA/dab_ctrl/ui_ctrl/scopes ==
  Bus Creator : BusCreator  Inputs=2
  Bus Creator1 : BusCreator  Inputs=2
  dab-tracking : Scope  NumInputPorts=2
      settings: ActiveDisplayYMinimum=-5.9234619140625  ActiveDisplayYMaximum=7.1295166015625  DataLoggingVariableName=ScopeData7
  u_ctrl_out_dab/i_ctrl_out_dab : Scope  NumInputPorts=2
      settings: ActiveDisplayYMinimum=-1.2812486231311795  ActiveDisplayYMaximum=1.531237608180616
  wires:
  Bus Creator1/1 -> dab-tracking/2
  Bus Creator/1 -> dab-tracking/1
  [i_ctrl_out_dab] -> u_ctrl_out_dab/i_ctrl_out_dab/2  "i_ctrl_out_dab"
  [i_out_pu_dab] -> Bus Creator1/2  "i_in_pu_dab"
  [uout_ref_pu_dab] -> Bus Creator/1  "uout_ref_pu_dab"
  [u_ctrl_out_dab] -> u_ctrl_out_dab/i_ctrl_out_dab/1  "u_ctrl_out_dab"
  [u_ctrl_out_dab] -> Bus Creator1/1  "u_ctrl_out_dab"
  [uout_pu_dab] -> Bus Creator/2  "uout_pu_dab"

== system dcdc_zvs_full_bridge/dab_modA/dcdc_with_galvanic_isolation/full-bridge-1/dclink ==
  CFi_dc1 : fl_lib/Electrical/Electrical Elements/Capacitor  c=CFi_dc1 F  r=RCFi_dc1_internal Ohm  g=0 1/Ohm  i_specify=off  i_priority=None  i=0 A  i_nominal_specify=off  i_nominal_value=1  i_nominal_unit=A  v_specify=off  v_priority=None  v=0 V  v_nominal_specify=off  v_nominal_value=1  v_nominal_unit=V  vc_specify=off  vc_priority=High  vc=0 V  vc_nominal_specify=off  vc_nominal_value=1  vc_nominal_unit=V
  Current Sensor : fl_lib/Electrical/Electrical Sensors/Current Sensor
  PS-Simulink Converter1 : nesl_utility/PS-Simulink Converter  PhysicalDomain=network_engine_domain  SubClassName=ps_output  LeftPortType=input  RightPortType=output  PseudoPeriodic=off  Frequencies=[]  VectorFormat=1-D array  Unit=A  AffineConversion=on
  PS-Simulink Converter4 : nesl_utility/PS-Simulink Converter  PhysicalDomain=network_engine_domain  SubClassName=ps_output  LeftPortType=input  RightPortType=output  PseudoPeriodic=off  Frequencies=[]  VectorFormat=1-D array  Unit=V  AffineConversion=on
  Voltage Sensor : fl_lib/Electrical/Electrical Sensors/Voltage Sensor
  udc(+) : PMIOPort  Side=Left
  Udc(+) : PMIOPort  Port=2  Side=Right
  udc(-) : PMIOPort  Port=3  Side=Left
  Udc(-) : PMIOPort  Port=4  Side=Right
  tag scope: CFi_dc_current=global, dab_voltage_input_modA=global
  wires:
  PS-Simulink Converter4/1 -> [dab_voltage_input_modA]  "dab_voltage_input_modA"
  PS-Simulink Converter1/1 -> [CFi_dc_current]  "CFi_dc_current"
  connections:
  Current Sensor/RConn1 -- PS-Simulink Converter1/LConn1
  PS-Simulink Converter4/LConn1 -- Voltage Sensor/RConn1
  Current Sensor/LConn1 -- CFi_dc1/RConn1
  Voltage Sensor/LConn1 -- Udc(+)/RConn1 -- CFi_dc1/LConn1 -- udc(+)/RConn1
  Current Sensor/RConn2 -- Udc(-)/RConn1 -- udc(-)/RConn1 -- Voltage Sensor/RConn2

== system dcdc_zvs_full_bridge/dab_modA/dcdc_with_galvanic_isolation/rectifier/dclink ==
  CFi_dc2 : fl_lib/Electrical/Electrical Elements/Capacitor  c=CFu_dc2 F  r=RCFu_dc2_internal Ohm  g=0 1/Ohm  i_specify=off  i_priority=None  i=0 A  i_nominal_specify=off  i_nominal_value=1  i_nominal_unit=A  v_specify=off  v_priority=None  v=0 V  v_nominal_specify=off  v_nominal_value=1  v_nominal_unit=V  vc_specify=off  vc_priority=High  vc=0 V  vc_nominal_specify=off  vc_nominal_value=1  vc_nominal_unit=V
  Current Sensor2 : fl_lib/Electrical/Electrical Sensors/Current Sensor
  PS-Simulink Converter6 : nesl_utility/PS-Simulink Converter  PhysicalDomain=network_engine_domain  SubClassName=ps_output  LeftPortType=input  RightPortType=output  PseudoPeriodic=off  Frequencies=[]  VectorFormat=1-D array  Unit=A  AffineConversion=on
  ui_measure : Subsystem
  udc(+) : PMIOPort  Side=Left
  udc(-) : PMIOPort  Port=2  Side=Left
  Udc(+) : PMIOPort  Port=3  Side=Right
  Udc(-) : PMIOPort  Port=4  Side=Right
  tag scope: CFi_dc2_current_modA=global
  wires:
  PS-Simulink Converter6/1 -> [CFi_dc2_current_modA]  "CFi_dc2_current_modA"
  connections:
  CFi_dc2/RConn1 -- Current Sensor2/LConn1
  PS-Simulink Converter6/LConn1 -- Current Sensor2/RConn1
  Current Sensor2/RConn2 -- udc(-)/RConn1 -- ui_measure/LConn2
  CFi_dc2/LConn1 -- udc(+)/RConn1 -- ui_measure/LConn1
  Udc(+)/RConn1 -- ui_measure/RConn1
  Udc(-)/RConn1 -- ui_measure/RConn2

== system dcdc_zvs_full_bridge/dab_modA/dcdc_with_galvanic_isolation/rectifier/rectifier_1 ==
  LFu_dc2_1 : fl_lib/Electrical/Electrical Elements/Inductor  l=LFu_dc2 H  r=RLFu_dc2 Ohm  g=1e-9 1/Ohm  i_specify=off  i_priority=None  i=0 A  i_nominal_specify=off  i_nominal_value=1  i_nominal_unit=A  v_specify=off  v_priority=None  v=0 V  v_nominal_specify=off  v_nominal_value=1  v_nominal_unit=V  i_L_specify=off  i_L_priority=High  i_L=0 A  i_L_nominal_specify=off  i_L_nominal_value=1  i_L_nominal_unit=A
  LFu_dc2_2 : fl_lib/Electrical/Electrical Elements/Inductor  l=LFu_dc2 H  r=RLFu_dc2 Ohm  g=1e-9 1/Ohm  i_specify=off  i_priority=None  i=0 A  i_nominal_specify=off  i_nominal_value=1  i_nominal_unit=A  v_specify=off  v_priority=None  v=0 V  v_nominal_specify=off  v_nominal_value=1  v_nominal_unit=V  i_L_specify=off  i_L_priority=High  i_L=0 A  i_L_nominal_specify=off  i_L_nominal_value=1  i_L_nominal_unit=A
  full_bridge_diode_rectifier_1 : full_bridge_diode_rectifier/full_bridge_diode_rectifier  Vf_diode_rectifier=0.35  Rdon_diode_rectifier=0.25e-3  Csnubber=Csnubber  Rsnubber=Rsnubber
  measurements_rectifier_output_1 : Subsystem
  u2(+) : PMIOPort  Side=Left
  udc(+) : PMIOPort  Port=2  Side=Right
  u2(-) : PMIOPort  Port=3  Side=Left
  udc(-) : PMIOPort  Port=4  Side=Right
  tag scope: diode_rectifier_bridge_1=global
  wires:
  full_bridge_diode_rectifier_1/1 -> [diode_rectifier_bridge_1]
  connections:
  measurements_rectifier_output_1/RConn2 -- LFu_dc2_2/LConn1
  measurements_rectifier_output_1/RConn1 -- LFu_dc2_1/LConn1
  measurements_rectifier_output_1/LConn1 -- full_bridge_diode_rectifier_1/RConn1
  measurements_rectifier_output_1/LConn2 -- full_bridge_diode_rectifier_1/RConn2
  u2(-)/RConn1 -- full_bridge_diode_rectifier_1/LConn2
  u2(+)/RConn1 -- full_bridge_diode_rectifier_1/LConn1
  udc(+)/RConn1 -- LFu_dc2_1/RConn1
  udc(-)/RConn1 -- LFu_dc2_2/RConn1

== system dcdc_zvs_full_bridge/dab_modA/dcdc_with_galvanic_isolation/rectifier/rectifier_2 ==
  LFu_dc2_1 : fl_lib/Electrical/Electrical Elements/Inductor  l=LFu_dc2 H  r=RLFu_dc2 Ohm  g=1e-9 1/Ohm  i_specify=off  i_priority=None  i=0 A  i_nominal_specify=off  i_nominal_value=1  i_nominal_unit=A  v_specify=off  v_priority=None  v=0 V  v_nominal_specify=off  v_nominal_value=1  v_nominal_unit=V  i_L_specify=off  i_L_priority=High  i_L=0 A  i_L_nominal_specify=off  i_L_nominal_value=1  i_L_nominal_unit=A
  LFu_dc2_2 : fl_lib/Electrical/Electrical Elements/Inductor  l=LFu_dc2 H  r=RLFu_dc2 Ohm  g=1e-9 1/Ohm  i_specify=off  i_priority=None  i=0 A  i_nominal_specify=off  i_nominal_value=1  i_nominal_unit=A  v_specify=off  v_priority=None  v=0 V  v_nominal_specify=off  v_nominal_value=1  v_nominal_unit=V  i_L_specify=off  i_L_priority=High  i_L=0 A  i_L_nominal_specify=off  i_L_nominal_value=1  i_L_nominal_unit=A
  full_bridge_diode_rectifier_1 : full_bridge_diode_rectifier/full_bridge_diode_rectifier  Vf_diode_rectifier=0.35  Rdon_diode_rectifier=0.25e-3  Csnubber=Csnubber  Rsnubber=Rsnubber
  measurements_rectifier_output_1 : Subsystem
  u2(+) : PMIOPort  Side=Left
  udc(+) : PMIOPort  Port=2  Side=Right
  u2(-) : PMIOPort  Port=3  Side=Left
  udc(-) : PMIOPort  Port=4  Side=Right
  tag scope: diode_rectifier_bridge_2=global
  wires:
  full_bridge_diode_rectifier_1/1 -> [diode_rectifier_bridge_2]
  connections:
  udc(-)/RConn1 -- LFu_dc2_2/RConn1
  udc(+)/RConn1 -- LFu_dc2_1/RConn1
  measurements_rectifier_output_1/RConn1 -- LFu_dc2_1/LConn1
  measurements_rectifier_output_1/RConn2 -- LFu_dc2_2/LConn1
  full_bridge_diode_rectifier_1/RConn1 -- measurements_rectifier_output_1/LConn1
  full_bridge_diode_rectifier_1/RConn2 -- measurements_rectifier_output_1/LConn2
  u2(-)/RConn1 -- full_bridge_diode_rectifier_1/LConn2
  u2(+)/RConn1 -- full_bridge_diode_rectifier_1/LConn1

== system dcdc_zvs_full_bridge/dab_modA/dab_ctrl/ui_ctrl/dab_ctrl/Vout Ctrl ==
  vout_ref : Inport
  vout : Inport  Port=2
  pi_ctrl : pi_ctrl/pi_ctrl  kp=kp_v_dab  ki=ki_v_dab  ts=ts_dab  lim_up=2  lim_down=-2
  ctrlv_out : Outport
  wires:
  vout_ref/1 -> pi_ctrl/1
  vout/1 -> pi_ctrl/2
  pi_ctrl/1 -> ctrlv_out/1

== system dcdc_zvs_full_bridge/dab_modA/dab_ctrl/ui_ctrl/dab_ctrl/current control ==
  i_out_dab_ref : Inport
  i_out_dab : Inport  Port=2
  i_out_dab_tracking : Scope  NumInputPorts=3
      settings: ActiveDisplayYMinimum=-0.71874108316637786  ActiveDisplayYMaximum=1.6339640481913458  DataLoggingVariableName=ScopeData12
  pi_ctrl : pi_ctrl/pi_ctrl  kp=kp_i_dab  ki=ki_i_dab  ts=ts_dab  lim_up=1  lim_down=-1
  i_ctrl_out : Outport
  wires:
  i_out_dab_ref/1 -> pi_ctrl/1, pi_ctrl/3, i_out_dab_tracking/1  "i_out_dab_ref"
  i_out_dab/1 -> pi_ctrl/2, i_out_dab_tracking/2  "i_out_dab"
  pi_ctrl/1 -> i_ctrl_out/1, i_out_dab_tracking/3  "i_dab_ctrl_out"
